simulink model "RetroalimentacionNoLineal_v2"  (R2026b)
settings: Solver=VariableStepAuto
values from neighbouring files (symbols this model uses):
  b_m = 2e-6    (= 2e-06)    [Pendulo_Invertido.m]
  b_theta = 1e-3    (= 0.001)    [Pendulo_Invertido.m]
  b_x = 0.10    (= 0.1)    [Pendulo_Invertido.m]
  g = 9.80665    [Pendulo_Invertido.m]
  Jm = 7.9e-6    (= 7.9e-06)    [Pendulo_Invertido.m]
  Jp = m2*l*l + I    (= 0.024)    [Pendulo_Invertido.m]
  kt = 0.0292    [Pendulo_Invertido.m]
  l = 0.30    (= 0.3)    [Pendulo_Invertido.m]
  M = m1+m2    (= 0.7)    [Pendulo_Invertido.m]
  m2 = 0.20    (= 0.2)    [Pendulo_Invertido.m]
  r = 0.010    (= 0.01)    [Pendulo_Invertido.m]    (also in barrer_pid_theta.m = T(T.Kp==o.Kp(a)&T.Kd==o.Kd(b)&T.Ki==ki,:))
settings Model: Creator=fedeb  LastModifiedBy=fedeb

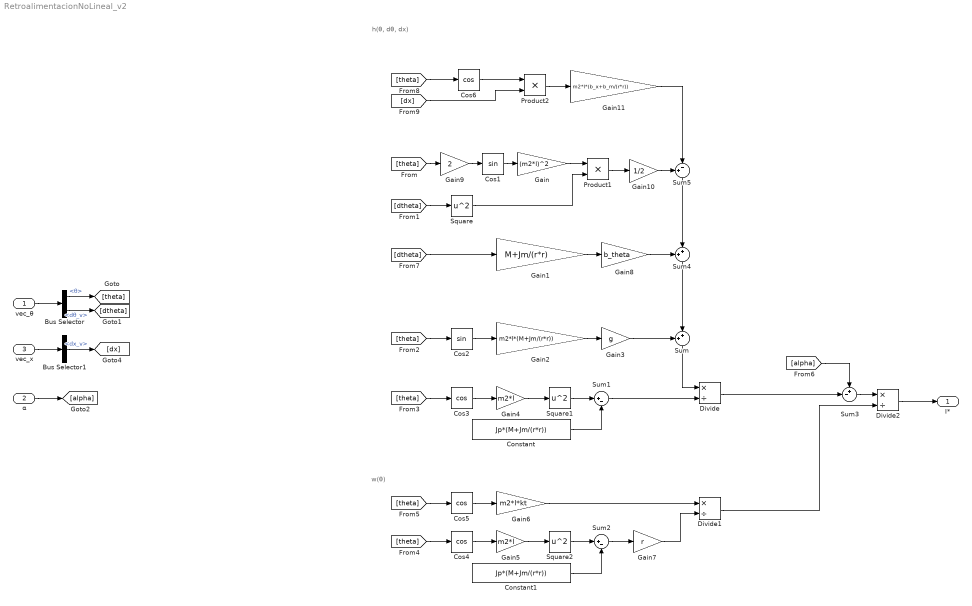
== system RetroalimentacionNoLineal_v2 ==
  note: h(θ, dθ, dx)
  note: w(θ)
  vec_θ : Inport
  α : Inport  Port=2
  vec_x : Inport  Port=3
  Bus Selector : BusSelector  OutputSignals=θ,dθ_v
  Bus Selector1 : BusSelector  OutputSignals=dx_v
  Constant : Constant  Value=Jp*(M+Jm/(r*r))
  Constant1 : Constant  Value=Jp*(M+Jm/(r*r))
  Cos1 : Trigonometry
  Cos2 : Trigonometry
  Cos{3..6} (4 alike) : Trigonometry  Operator=cos
  Divide : Product  Inputs=*/
  Divide1 : Product  Inputs=*/
  Divide2 : Product  Inputs=*/
  Gain : Gain  Gain=(m2*l)^2
  Gain1 : Gain  Gain=M+Jm/(r*r)
  Gain10 : Gain  Gain=1/2
  Gain11 : Gain  Gain=m2*l*(b_x+b_m/(r*r))
  Gain2 : Gain  Gain=m2*l*(M+Jm/(r*r))
  Gain3 : Gain  Gain=g
  Gain4 : Gain  Gain=m2*l
  Gain5 : Gain  Gain=m2*l
  Gain6 : Gain  Gain=m2*l*kt
  Gain7 : Gain  Gain=r
  Gain8 : Gain  Gain=b_theta
  Gain9 : Gain  Gain=2
  Product1 : Product
  Product2 : Product
  Square : Math  Operator=square
  Square1 : Math  Operator=square
  Square2 : Math  Operator=square
  Sum : Sum  Inputs=++|
  Sum1 : Sum  Inputs=|+-
  Sum2 : Sum  Inputs=|+-
  Sum3 : Sum  Inputs=+-|
  Sum4 : Sum  Inputs=++|
  Sum5 : Sum  Inputs=+-|
  Ⅰ* : Outport
  wires:
  Sum/1 -> Divide/1
  Square/1 -> Product1/2
  Sum3/1 -> Divide2/1
  Gain4/1 -> Square1/1
  Cos5/1 -> Gain6/1
  Constant/1 -> Sum1/2
  Sum1/1 -> Divide/2
  Gain2/1 -> Gain3/1
  Divide2/1 -> Ⅰ*/1
  Square1/1 -> Sum1/1
  vec_θ/1 -> Bus Selector/1
  Gain/1 -> Product1/1
  [alpha] -> Sum3/1
  Gain3/1 -> Sum/1
  Bus Selector/1 -> [theta]  "<θ>"
  [theta] -> Cos3/1
  Divide/1 -> Sum3/2
  α/1 -> [alpha]
  Cos3/1 -> Gain4/1
  Gain6/1 -> Divide1/1
  [theta] -> Gain9/1
  Bus Selector/2 -> [dtheta]  "<dθ_v>"
  [dtheta] -> Square/1
  [theta] -> Cos2/1
  [theta] -> Cos5/1
  Divide1/1 -> Divide2/2
  Cos4/1 -> Gain5/1
  [theta] -> Cos4/1
  Square2/1 -> Sum2/1
  Gain5/1 -> Square2/1
  Sum2/1 -> Gain7/1
  Constant1/1 -> Sum2/2
  Gain7/1 -> Divide1/2
  vec_x/1 -> Bus Selector1/1
  Bus Selector1/1 -> [dx]  "<dx_v>"
  Sum4/1 -> Sum/2
  Sum5/1 -> Sum4/2
  Cos2/1 -> Gain2/1
  Gain1/1 -> Gain8/1
  Gain8/1 -> Sum4/1
  [dtheta] -> Gain1/1
  Gain9/1 -> Cos1/1
  Cos1/1 -> Gain/1
  Product1/1 -> Gain10/1
  Gain10/1 -> Sum5/1
  [theta] -> Cos6/1
  Cos6/1 -> Product2/1
  [dx] -> Product2/2
  Product2/1 -> Gain11/1
  Gain11/1 -> Sum5/2
